simulink model "LKS"  (R2025b)
settings: Solver=VariableStepAuto  StartTime=0.0  StopTime=200  RelTol=1e-3
values from neighbouring files (symbols this model uses):
  v = 30    [LKS_challenge.m]
undefined symbols (not defined in the file or in its folder): A, driving, w
libraries: drivingscenarioandsensors x2, robotmobilelib x1, slpidlib x1, sim3dlib x1, sim3dautolib x1
settings Model: Creator=dell  LastModifiedBy=dell

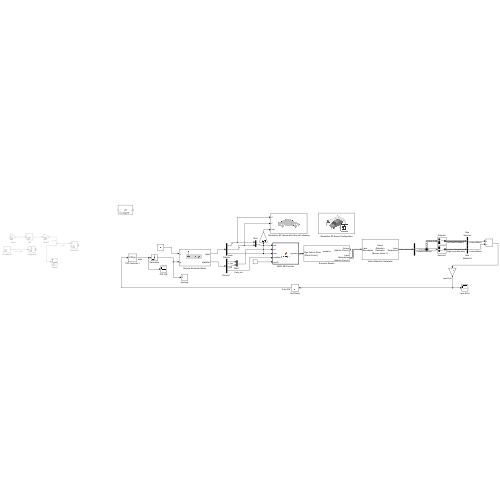
[thumbnail: Simulink's stored preview of the top-level diagram]
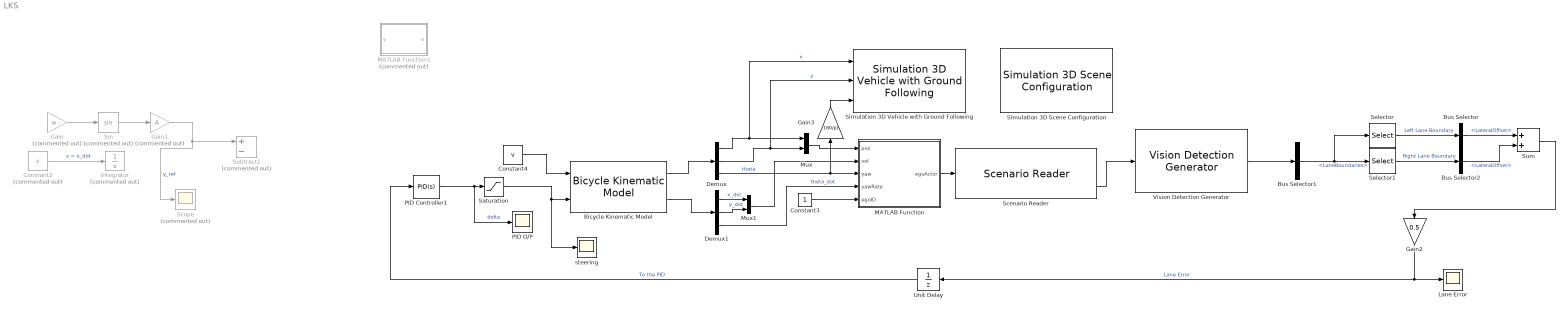
== system LKS ==
  Bicycle Kinematic Model : robotmobilelib/Bicycle Kinematic Model  VehicleInputs=Vehicle Speed & Steering Angle  WheelBase=L  VehicleSpeedRange=[-inf inf]  MaxSteeringAngle=pi/4  InitialState=[8.9696932066214; 14.9560053468342; 0.01]  SimulateUsing=Interpreted execution
  Bus Selector : BusSelector  OutputSignals=LateralOffset
  Bus Selector1 : BusSelector  OutputSignals=LaneBoundaries
  Bus Selector2 : BusSelector  OutputSignals=LateralOffset
  Constant2 : Constant  Commented=on  Value=v
  Constant3 : Constant
  Constant4 : Constant  Value=v
  Demux : Demux  Outputs=3
  Demux1 : Demux  Outputs=3
  Gain : Gain  Commented=on  Gain=w
  Gain1 : Gain  Commented=on  Gain=A
  Gain2 : Gain  Gain=0.5
  Gain3 : Gain  Gain=180/pi
  Integrator : Integrator  Commented=on
  Lane Error : Scope
  MATLAB Function : MATLAB Function  TreatAsAtomicUnit=on
  MATLAB Function1 : MATLAB Function  Commented=on  TreatAsAtomicUnit=on
  Mux : Mux  Inputs=2
  Mux1 : Mux  Inputs=2
  PID Controller1 : slpidlib/PID Controller  Controller=PID  Form=Parallel  TimeDomain=Continuous-time  UseExternalTs=off  SampleTime=-1  IntegratorMethod=Forward Euler  FilterMethod=Forward Euler  ControllerParametersSource=internal  P=1  I=0  UseKiTs=off  D=0  UseExternalDerivativeSource=off  N=100  UseFilter=on  TunerSelectOption=Transfer Function Based (PID Tuner App)  InitialConditionSource=internal  InitialConditionForIntegrator=0  InitialConditionForFilter=0  DifferentiatorICPrevScaledInput=0  ExternalReset=none  TrackingMode=off  Kt=1  LimitOutput=off  SatLimitsSource=internal  UpperSaturationLimit=inf  LowerSaturationLimit=-inf  LinearizeAsGain=on  AntiWindupMode=none  Kb=1  LimitIntegrator=off  UpperIntegratorSaturationLimit=inf  LowerIntegratorSaturationLimit=-inf  POutMin=[]  POutMax=[]  IOutMin=[]  IOutMax=[]  DOutMin=[]  DOutMax=[]  NOutMin=[]  NOutMax=[]  SumOutMin=[]  SumOutMax=[]  SaturationOutMin=[]  SaturationOutMax=[]  PParamMin=[]  PParamMax=[]  IParamMin=[]  IParamMax=[]  DParamMin=[]  DParamMax=[]  NParamMin=[]  NParamMax=[]  KbParamMin=[]  KbParamMax=[]  KtParamMin=[]  KtParamMax=[]  KbOutMin=[]  KbOutMax=[]  KtOutMin=[]  KtOutMax=[]  IntegratorOutMin=[]  IntegratorOutMax=[]  FilterOutMin=[]  FilterOutMax=[]  SumI1OutMin=[]  SumI1OutMax=[]  SumI2OutMin=[]  SumI2OutMax=[]  SumI3OutMin=[]  SumI3OutMax=[]  SumI4OutMin=[]  SumI4OutMax=[]  SumDOutMin=[]  SumDOutMax=[]  DifferentiatorOutMin=[]  DifferentiatorOutMax=[]  FilterDiffOutCoefMin=[]  FilterDiffOutCoefMax=[]  ReciprocalOutMin=[]  ReciprocalOutMax=[]  SumDenOutMin=[]  SumDenOutMax=[]  SumNumOutMin=[]  SumNumOutMax=[]  DivideOutMin=[]  DivideOutMax=[]  UdiffTsProdOutMin=[]  UdiffTsProdOutMax=[]  NTsProdOutMin=[]  NTsProdOutMax=[]  UintegralTsProdOutMin=[]  UintegralTsProdOutMax=[]  UngainTsProdOutMin=[]  UngainTsProdOutMax=[]  ClampingZeroOutDataTypeStr=Inherit: Inherit via back propagation  ClampingZeroOutMin=[]  ClampingZeroOutMax=[]  FilterDenConstantOutDataTypeStr=Inherit: Inherit via back propagation  FilterDenConstantOutMin=[]  FilterDenConstantOutMax=[]  PCopyOutDataTypeStr=Inherit: Inherit via back propagation  PCopyOutMin=[]  PCopyOutMax=[]  NCopyOutDataTypeStr=Inherit: Inherit via back propagation  NCopyOutMin=[]  NCopyOutMax=[]  IntegratorContinuousStateAttributes=''  IntegratorStateMustResolveToSignalObject=off  IntegratorRTWStateStorageClass=Auto  FilterContinuousStateAttributes=''  FilterStateMustResolveToSignalObject=off  FilterRTWStateStorageClass=Auto  ParallelPVariant=InternalParameters  IdealPVariant=Disabled  IVariant=InternalParameters  DVariant=InternalParameters  IntegratorVariant=Continuous  SatVariant=Disabled  AWVariant=Passthrough  PCopyVariant=Disabled  TRVariant=Disabled  FdbkBlocksVariant=Forward  IdealPFdbkVariant=Disabled  SatFdbkVariant=Disabled  DerivativeFilterVariant=ContFilter  NVariant=InternalParameters  NCopyVariant=Disabled  FilterICVariant=InternalICsFilter  IntegratorICVariant=InternalICs  ExternalResetVariant=Disabled  TRSumVariant=Passthrough  SumFdbkVariant=Disabled  SumVariant=Sum_PID  TsampFilterVariant=InternalTs  TsampNgainVariant=Passthrough  TsampIntegralVariant=Disabled_SignalSpec  ExternalSaturationOutDataTypeStr=Inherit: Same as second input  DerivativeSourceVariant=ErrorSignal  PreIntVariant=InternalPreInt
  PID O/P : Scope
      settings: ActiveDisplayYMinimum=-1.6564637123098991  ActiveDisplayYMaximum=2.8019464436672239  DataLoggingVariableName=ScopeData2
  Saturation : Saturate  UpperLimit=0.3  LowerLimit=-0.3
  Scenario Reader : drivingscenarioandsensors/Scenario Reader  ScenarioSource=From file  ScenarioFileName=C:\Users\dell\Desktop\New folder (3)\challenge\scenario.mat  ScenarioVariableName=scenario  OutputCoordinateSystem=Vehicle coordinates  EgoVehicleSource=Input port  EgoVehicleActorID=1  OrientVehiclesOnRoad=off  OutputEgoVehiclePose=off  OutputEgoVehicleState=off  SampleTime=0.1  LaneBoundaryOutput=Ego vehicle lane boundaries  LaneBoundaryDistance=0:1:50  LaneBoundaryLocation=Center of lane markings  BusNameSource=Auto  BusName=BusActors  BusNumActorsSource=Scenario  BusNumActors=100  BusName2Source=Auto  BusName2=BusLaneBoundaries  BusNumLaneBoundariesSource=Scenario  BusNumLaneBoundaries=10  BusName3Source=Auto  BusName3=BusEgoActor  BusName4Source=Auto  BusName4=BusEgoState  ShowCoordinateLabels=on  SimulateUsing=Interpreted execution
  Scope : Scope  Commented=on
      settings: ActiveDisplayYMinimum=-2.4999902591305236  ActiveDisplayYMaximum=2.4999982605203397
  Selector : Selector  InputPortWidth=2  IndexOptions=Index vector (dialog)  Indices=1  OutputSizes=1
  Selector1 : Selector  InputPortWidth=2  IndexOptions=Index vector (dialog)  Indices=2  OutputSizes=1
  Simulation 3D Scene Configuration : sim3dlib/Simulation 3D Scene Configuration  Priority=0  ProjectFormat=Default Scenes  SceneDesc=Curved road  ProjectName=C:\Program Files\MATLAB\R2025b\toolbox\shared\sim3d_projects\automotive_project_windows\UE\WindowsNoEditor\VehicleSimulation.exe  ScenePath=/Game/Maps/HwStrght  EnableOpenDRIVE=off  vehTagList={'Custom';'Scene Origin';'SimulinkVehicle1'}  vehTag=Scene Origin  AttachedCameraRelativeTranslation=[0 0 0]  FreeCameraDefaultInitialTranslation=[-6, 0, 2]  AttachedCameraRelativeRotation=[0 0 0]  FreeCameraDefaultInitialRotation=[0, -15, 0]  ViewpointName=Custom  FreeCameraInitialTranslation=[0, 0, 0]  ViewpointTranslation=[0 0 0]  FreeCameraInitialRotation=[0, 0, 0]  ViewpointRotation=[0 0 0]  OpVisEn=off  Ts=1/60  EnableWindow=on  EnableRemoteAccess=off  EnableWeather=off  SunAzimuth=90  SunAltitude=40.0  EnableGeospatialSun=off  Latitude=0  Longitude=0  Date=2023-01-01  Time=10:30:00  GeoTimeZone=-5.0  SunDaylightSaving=off  wind=1  clouds=10  EnableVolumetricClouds=off  CloudCoverage=0  CloudAltitude=6  fog=0  rain=0  RaindropsEffect=off  SnowDensity=0  EnableGeospatial=off  TilesetSource=Earth terrain  UseTrueOrigin=off  OriginHeight=200  OriginLatitude=40.744652  OriginLongitude=-73.988864  MapStyle=Aerial  AdditionalAssetIDs=[]  UseAdvancedSunSky=off  SolarTime=11  TimeZone=-5  Day=21  Month=9  Year=2022  UseDaylightSavingTime=on  DSTStartDay=10  DSTStartMonth=3  DSTEndDay=3  DSTEndMonth=11  DSTSwitchHour=2  sensorTag=MainCamera1  sensorId=1  sensorName=MainCamera1  mountLoc=Origin  offsetFlag=off  tmountOffset=[0, 0, 0]  rmountOffset=[0, 0, 0]  HorizontalResolution=1280  VerticalResolution=720  HorizontalFOV=60  mountPoint=[0 0 0]  mountOrientation=[0 0 0]  aMode=3  ID=1  GeoTrigger=Inactive  ViewNameList={'Custom'}  ViewTranslationList={'[0 0 0]'}  ViewRotationList={'[0 0 0]'}
      settings: LibrarySourceBlock=drivingsim3d/Simulation 3D Scene Configuration
  Simulation 3D Vehicle with Ground Following : sim3dautolib/Simulation 3D Vehicle with Ground Following  Priority=-1  PassVehMesh=Sedan  MeshPath=/MathWorksAutomotiveContent/Vehicles/Muscle/Meshes/SK_MuscleCar.SK_MuscleCar  TrackWidth=1.9  WheelBase=3  WheelRadius=0.35  VehColor=Red  CoordinateSystem=ISO8855  InitialPos=[8.9696932066214, 14.9560053468342, 0]  InitialRot=[0, 0, -3.84]  ActorName=SimulinkVehicle1  SampleTime=-1  ActorType=SimulinkVehicle  ID=1  aMode=3  ActorTag=SimulinkVehicle1  CoordinateScheme=0  VehLightsControl=off  HeadlightColor=[ 1, 1, 1 ]  HighBeamIntensity=100000  LowBeamIntensity=60000  HighBeamConeAngle=70  LowBeamConeAngle=70  LeftHeadlightOrientation=[ 0, 0 ]  RightHeadlightOrientation=[ 0, 0 ]  BrakelightIntensity=500  ReverselightIntensity=500  SignallightIntensity=500  SignallightPeriod=1  SignalPulseWidth=50  TransformOutportEnabled=off
      settings: LibrarySourceBlock=drivingsim3d/Simulation 3D Vehicle with Ground Following
  Sin : Trigonometry  Commented=on
  Subtract1 : Sum  Commented=on  Inputs=+-
  Sum : Sum
  Unit Delay : UnitDelay  SampleTime=0.1  HasFrameUpgradeWarning=on
  Vision Detection Generator : drivingscenarioandsensors/Vision Detection Generator  SensorIndex=1  DetectorOutput=Lanes only  UpdateInterval=0.1  LaneUpdateInterval=0.1  SensorLocation=[ 1.9, 0 ]  Height=1.1  Yaw=0  Pitch=1  Roll=0  BusNameSource=Auto  BusName=BusObjectDetections  BusName2Source=Auto  BusName2=BusLaneDetections  MaxNumDetectionsSource=Property  MaxNumDetections=50  MaxNumLanesSource=Property  MaxNumLanes=2  DetectionCoordinates=Ego Cartesian  SimulateUsing=Interpreted execution  MaxRange=150  BoundingBoxAccuracy=5  ProcessNoiseIntensity=5  MaxSpeed=100  MaxAllowedOcclusion=0.5  MinObjectImageSize=[ 15, 15 ]  DetectionProbability=0.9  FalsePositivesPerImage=0.1  MinLaneImageSize=[ 20, 3 ]  LaneBoundaryAccuracy=3  HasNoise=on  InitialSeedSource=Repeatable  InitialSeed=0  UsedSeed=driving.internal.SimulinkUtilities.seedManager(gcb)  ActorProfilesSource=From Scenario Reader block  ActorProfilesParameters=driving.internal.ActorProfilesParameters  ActorProfilesExpression=struct( 'ClassID', 0, 'Length', 4.7, 'Width', 1.8, 'Height', 1.4, 'OriginOffset', [ -1.35, 0, 0 ] )  Intrinsics=driving.internal.cameraIntrinsics
  steering : Scope
      settings: ActiveDisplayYMinimum=-0.493305776695152  ActiveDisplayYMaximum=0.60004193717392751  DataLoggingVariableName=ScopeData5
  wires:
  Constant2/1 -> Integrator/1  "v = x_dot"
  Gain/1 -> Sin/1
  Sin/1 -> Gain1/1
  PID Controller1/1 -> PID O/P/1, Saturation/1  "delta"
  Bicycle Kinematic Model/1 -> Demux/1
  Saturation/1 -> Bicycle Kinematic Model/2, steering/1
  Bicycle Kinematic Model/2 -> Demux1/1
  MATLAB Function/1(egoActor) -> Scenario Reader/1
  Demux1/2 -> Mux1/2  "y_dot"
  Mux1/1 -> MATLAB Function/2(vel)
  Demux/3 -> Gain3/1, MATLAB Function/3(yaw)  "theta"
  Demux1/3 -> MATLAB Function/4(yawRate)  "theta_dot"
  Constant3/1 -> MATLAB Function/5(egoID)
  Gain1/1 -> Subtract1/1, Scope/1  "y_ref"
  Constant4/1 -> Bicycle Kinematic Model/1
  Demux1/1 -> Mux1/1  "x_dot"
  Mux/1 -> MATLAB Function/1(pos)
  Demux/1 -> Simulation 3D Vehicle with Ground Following/1, Mux/1  "x"
  Demux/2 -> Mux/2, Simulation 3D Vehicle with Ground Following/2  "y"
  Scenario Reader/2 -> Vision Detection Generator/1
  Selector/1 -> Bus Selector/1  "Left Lane Boundary"
  Selector1/1 -> Bus Selector2/1  "Right Lane Boundary"
  Bus Selector/1 -> Sum/1  "<LateralOffset>"
  Bus Selector2/1 -> Sum/2  "<LateralOffset>"
  Sum/1 -> Gain2/1
  Gain2/1 -> Lane Error/1, Unit Delay/1  "Lane Error"
  Unit Delay/1 -> PID Controller1/1  "To the PID"
  Vision Detection Generator/1 -> Bus Selector1/1
  Bus Selector1/1 -> Selector/1, Selector1/1  "<LaneBoundaries>"
  Gain3/1 -> Simulation 3D Vehicle with Ground Following/3

== matlab function LKS/MATLAB Function1 ==
  data: u input; y output
function y = safeError(u)
    if isnan(u) || isinf(u)
        y = 0;
    else
        y = u;
    end
end

== matlab function LKS/MATLAB Function ==
  data: pos input size=2; vel input size=2; yaw input; yawRate input; egoID input; egoActor output Bus: EgoVehiclePoseBus
function egoActor = packEgo(pos,vel,yaw,yawRate,egoID)

egoActor = struct(...
    'ActorID',egoID,...
    'Position', [pos(1) pos(2) 0], ...
    'Velocity', [vel(1) vel(2) 0], ...
    'Roll', 0, ...
    'Pitch', 0, ...
    'Yaw', rad2deg(yaw), ...
    'AngularVelocity', [0 0 rad2deg(yawRate)]);

end
